simulink model "VRFB_lypunov_observer_model"  (R2024a)
settings: Solver=VariableStepAuto  StartTime=0.0  StopTime=10.0  RelTol=1e-3
undefined symbols (not defined in the file): c_V, d, E_neg, E_pos, E_T_23, E_T_34, E_T_45, eff_coulomb, F, g_neg, g_pos, gamma, H_init, k2, k3, k4, k5, kox, l, mu_init, R, S, T, u_upper_bound, Vc, Vt, x_real_init, z_13_low, z_13_up, z_24_low, z_24_up, z_hat_init
settings Model: Creator=DHADUKHA  LastModifiedBy=DHADUKHA

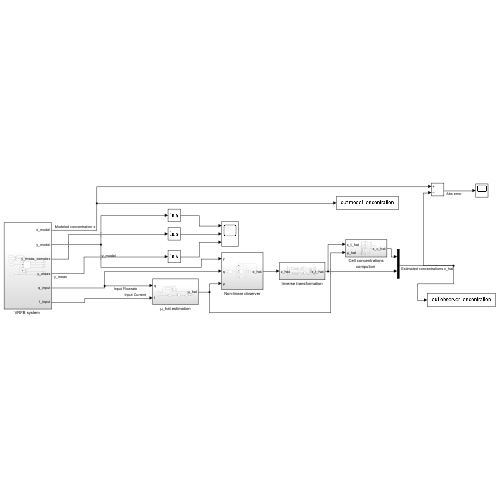
[thumbnail: Simulink's stored preview of the top-level diagram]
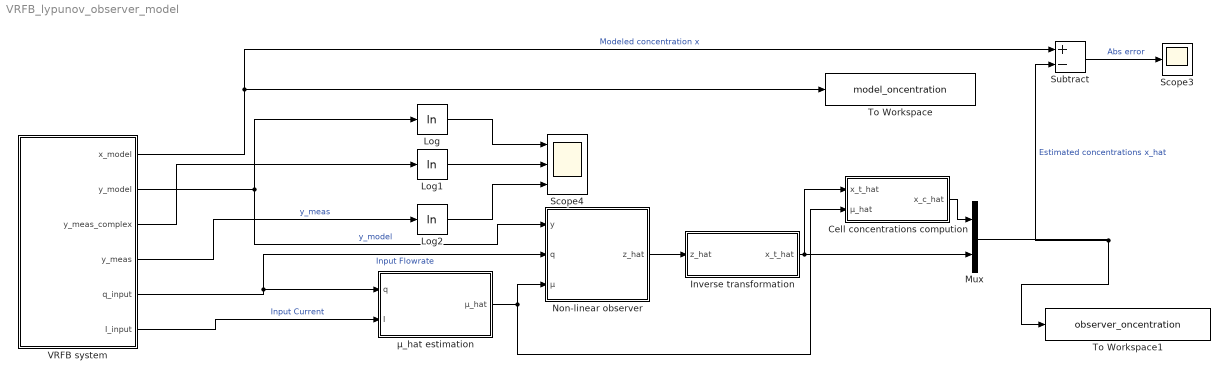
== system VRFB_lypunov_observer_model ==
  "Cell concentrations compution " : Subsystem
  "Inverse transformation " : Subsystem
  Log : Math  Operator=log
  Log1 : Math  Operator=log
  Log2 : Math  Operator=log
  Mux : Mux  Inputs=2
  "Non-linear observer " : Subsystem
  Scope3 : Scope
  Scope4 : Scope  NumInputPorts=3
  Subtract : Sum  Inputs=+-
  To Workspace : ToWorkspace  VariableName=model_oncentration  SaveFormat=Structure With Time  SampleTime=-1
  To Workspace1 : ToWorkspace  VariableName=observer_oncentration  SaveFormat=Structure With Time  SampleTime=-1
  "VRFB system " : Subsystem
  "µ_hat estimation " : Subsystem
  wires:
  "VRFB system "/5(q_input) -> "Non-linear observer "/2(q), "µ_hat estimation "/1(q)  "Input Flowrate"
  "VRFB system "/3(y_meas_complex) -> Log1/1
  "VRFB system "/1(x_model) -> Subtract/1, To Workspace/1  "Modeled concentration x"
  "VRFB system "/6(I_input) -> "µ_hat estimation "/2(I)  "Input Current"
  "VRFB system "/4(y_meas) -> Log2/1  "y_meas"
  "VRFB system "/2(y_model) -> "Non-linear observer "/1(y), Log/1  "y_model"
  Log1/1 -> Scope4/2
  Log/1 -> Scope4/1
  Log2/1 -> Scope4/3
  "µ_hat estimation "/1(µ_hat) -> "Non-linear observer "/3(µ), "Cell concentrations compution "/2(µ_hat)
  Subtract/1 -> Scope3/1  "Abs error"
  "Non-linear observer "/1(z_hat) -> "Inverse transformation "/1(z_hat)
  "Inverse transformation "/1(x_t_hat) -> "Cell concentrations compution "/1(x_t_hat), Mux/2
  "Cell concentrations compution "/1(x_c_hat) -> Mux/1
  Mux/1 -> Subtract/2, To Workspace1/1  "Estimated concentrations x_hat"

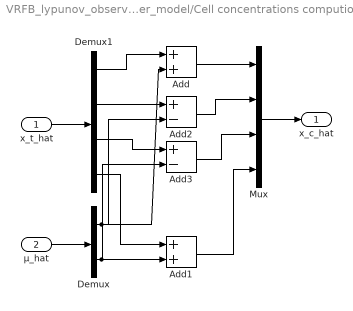
== system VRFB_lypunov_observer_model/Cell concentrations compution  ==
  x_t_hat : Inport
  µ_hat : Inport  Port=2
  Add : Sum
  Add1 : Sum
  Add2 : Sum  Inputs=+-
  Add3 : Sum  Inputs=+-
  Demux : Demux  Outputs=2
  Demux1 : Demux
  Mux : Mux
  x_c_hat : Outport
  wires:
  Demux1/4 -> Add1/1
  x_t_hat/1 -> Demux1/1
  Demux1/3 -> Add3/1
  µ_hat/1 -> Demux/1
  Demux/2 -> Add3/2, Add1/2
  Demux1/2 -> Add2/1
  Demux1/1 -> Add/1
  Demux/1 -> Add/2, Add2/2
  Add/1 -> Mux/1
  Add2/1 -> Mux/2
  Add3/1 -> Mux/3
  Add1/1 -> Mux/4
  Mux/1 -> x_c_hat/1

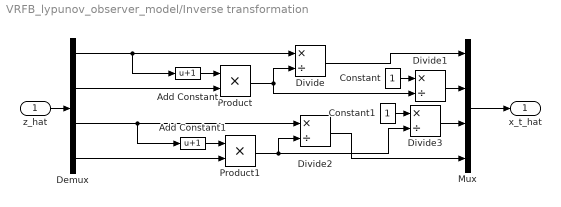
== system VRFB_lypunov_observer_model/Inverse transformation  ==
  z_hat : Inport
  Add Constant : Bias  Bias=1  SaturateOnIntegerOverflow=off
  Add Constant1 : Bias  Bias=1  SaturateOnIntegerOverflow=off
  Constant : Constant
  Constant1 : Constant
  Demux : Demux
  Divide{,1..3} (4 alike) : Product  Inputs=*/
  Mux : Mux
  Product : Product
  Product1 : Product
  x_t_hat : Outport
  wires:
  z_hat/1 -> Demux/1
  Demux/1 -> Add Constant/1, Divide/1
  Add Constant/1 -> Product/1
  Demux/2 -> Product/2
  Product/1 -> Divide1/2, Divide/2
  Mux/1 -> x_t_hat/1
  Divide/1 -> Mux/1
  Constant/1 -> Divide1/1
  Divide1/1 -> Mux/2
  Constant1/1 -> Divide3/1
  Product1/1 -> Divide2/2, Divide3/2
  Demux/4 -> Product1/2
  Add Constant1/1 -> Product1/1
  Demux/3 -> Divide2/1, Add Constant1/1
  Divide3/1 -> Mux/3
  Divide2/1 -> Mux/4

== system VRFB_lypunov_observer_model/Non-linear observer  ==
  y : Inport
  q : Inport  Port=2
  µ : Inport  Port=3
  Integrator : Integrator  InitialCondition=z_hat_init
  M(z_hat) : Subsystem
  Plus : Sum  Inputs=+++
  "f(z_hat, u)" : Subsystem
  "g(z_hat, y, u)" : Subsystem
  "u " : Subsystem
  z_hat : Outport
  wires:
  "f(z_hat, u)"/1(f) -> Plus/1
  "g(z_hat, y, u)"/1(g) -> Plus/2
  M(z_hat)/1(M) -> Plus/3
  Plus/1 -> Integrator/1  "z_hat_dot"
  Integrator/1 -> M(z_hat)/1(z_hat), "g(z_hat, y, u)"/1(z_hat), "f(z_hat, u)"/1(z_hat), z_hat/1
  q/1 -> "u "/1(q)
  "u "/1(u) -> M(z_hat)/2(u), "g(z_hat, y, u)"/3(u), "f(z_hat, u)"/2(u)
  y/1 -> "g(z_hat, y, u)"/2(y)
  µ/1 -> "u "/2(µ)

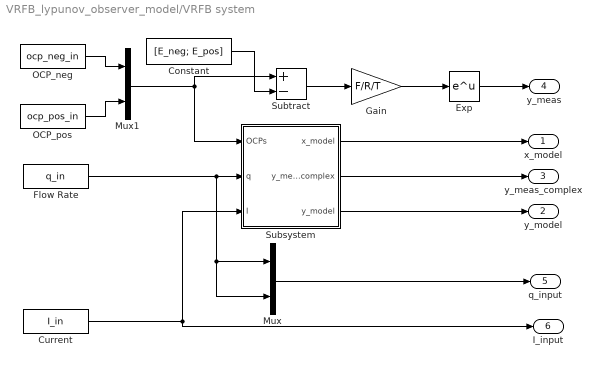
== system VRFB_lypunov_observer_model/VRFB system  ==
  Constant : Constant  Value=[E_neg; E_pos]
  Current : FromWorkspace  VariableName=I_in  SampleTime=1  OutputAfterFinalValue=Holding final value
  Exp : Math  OutputSignalType=real
  Flow Rate : FromWorkspace  VariableName=q_in  SampleTime=1  OutputAfterFinalValue=Holding final value
  Gain : Gain  Gain=F/R/T
  Mux : Mux  Inputs=2
  Mux1 : Mux  Inputs=2
  OCP_neg : FromWorkspace  VariableName=ocp_neg_in  SampleTime=1  OutputAfterFinalValue=Holding final value
  OCP_pos : FromWorkspace  VariableName=ocp_pos_in  SampleTime=1  OutputAfterFinalValue=Holding final value
  Subsystem : Subsystem
  Subtract : Sum  Inputs=+-
  x_model : Outport
  y_model : Outport  Port=2
  y_meas_complex : Outport  Port=3
  y_meas : Outport  Port=4
  q_input : Outport  Port=5
  I_input : Outport  Port=6
  wires:
  Subsystem/2(y_meas_complex) -> y_meas_complex/1
  Mux1/1 -> Subtract/1, Subsystem/1(OCPs)
  OCP_neg/1 -> Mux1/1
  Subsystem/1(x_model) -> x_model/1
  Flow Rate/1 -> Mux/1, Mux/2, Subsystem/2(q)
  Subtract/1 -> Gain/1
  OCP_pos/1 -> Mux1/2
  Current/1 -> Subsystem/3(I), I_input/1
  Constant/1 -> Subtract/2
  Subsystem/3(y_model) -> y_model/1
  Mux/1 -> q_input/1
  Gain/1 -> Exp/1
  Exp/1 -> y_meas/1

== system VRFB_lypunov_observer_model/µ_hat estimation  ==
  q : Inport
  I : Inport  Port=2
  Constant : Constant  Value=-(1/Vc+1/Vt)
  Gain : Gain  Gain=1/(F*Vc)
  Integrator : Integrator  InitialCondition=mu_init
  Plus : Sum
  Product : Product  Inputs=3
  µ_hat : Outport
  wires:
  I/1 -> Gain/1
  Gain/1 -> Plus/2
  q/1 -> Product/1
  Constant/1 -> Product/2
  Integrator/1 -> Product/3, µ_hat/1
  Product/1 -> Plus/1
  Plus/1 -> Integrator/1  "µ_dot_hat"

== system VRFB_lypunov_observer_model/Non-linear observer /M(z_hat) ==
  z_hat : Inport
  u : Inport  Port=2
  Constant1 : Constant  Value=[z_13_low; z_24_low; z_13_low; z_24_low]  VectorParams1D=off
  Constant2 : Constant  Value=[z_13_up; z_24_up; z_13_up; z_24_up]  VectorParams1D=off
  Gain : Gain  Gain=-gamma
  MATLAB Function : MATLAB Function  TreatAsAtomicUnit=on
  P-Matrix [4,4] : Subsystem
  Product : Product  Inputs=3  Multiplication=Matrix(*)
  "r(z_hat) " : Subsystem
  M : Outport
  wires:
  u/1 -> P-Matrix [4,4]/1(u)
  z_hat/1 -> MATLAB Function/1(z), "r(z_hat) "/1(z_hat)
  Constant2/1 -> MATLAB Function/3(z_max)
  Constant1/1 -> MATLAB Function/2(z_min)
  Product/1 -> Gain/1
  Gain/1 -> M/1
  P-Matrix [4,4]/1(P) -> Product/1
  MATLAB Function/1(drdz) -> Product/2
  "r(z_hat) "/1(r) -> Product/3

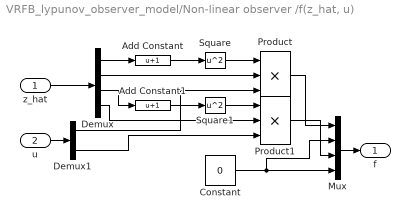
== system VRFB_lypunov_observer_model/Non-linear observer /f(z_hat, u) ==
  z_hat : Inport
  u : Inport  Port=2
  Add Constant : Bias  Bias=1  SaturateOnIntegerOverflow=off
  Add Constant1 : Bias  Bias=1  SaturateOnIntegerOverflow=off
  Constant : Constant  Value=0
  Demux : Demux
  Demux1 : Demux  Outputs=2
  Mux : Mux
  Product : Product  Inputs=3
  Product1 : Product  Inputs=3
  Square : Math  Operator=square
  Square1 : Math  Operator=square
  f : Outport
  wires:
  z_hat/1 -> Demux/1
  Mux/1 -> f/1
  Constant/1 -> Mux/2, Mux/4
  u/1 -> Demux1/1
  Demux/1 -> Add Constant/1
  Add Constant/1 -> Square/1
  Square/1 -> Product/1
  Demux1/1 -> Product/3
  Demux/2 -> Product/2
  Add Constant1/1 -> Square1/1
  Square1/1 -> Product1/1
  Demux/4 -> Product1/2
  Demux1/2 -> Product1/3
  Demux/3 -> Add Constant1/1
  Product1/1 -> Mux/3
  Product/1 -> Mux/1

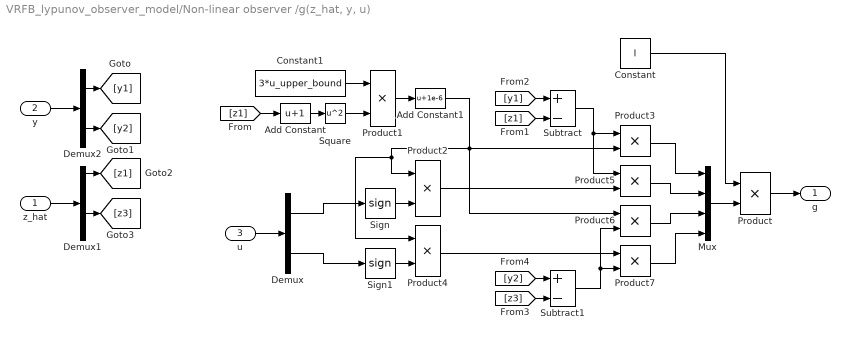
== system VRFB_lypunov_observer_model/Non-linear observer /g(z_hat, y, u) ==
  z_hat : Inport
  y : Inport  Port=2
  u : Inport  Port=3
  Add Constant : Bias  Bias=1  SaturateOnIntegerOverflow=off
  Add Constant1 : Bias  Bias=1e-6  SaturateOnIntegerOverflow=off
  Constant : Constant  Value=l
  Constant1 : Constant  Value=3*u_upper_bound
  Demux : Demux  Outputs=2
  Demux1 : Demux
  Demux2 : Demux  Outputs=2
  Mux : Mux
  Product{,1..7} (8 alike) : Product
  Sign : Signum
  Sign1 : Signum
  Square : Math  Operator=square
  Subtract : Sum  Inputs=+-
  Subtract1 : Sum  Inputs=+-
  g : Outport
  wires:
  u/1 -> Demux/1
  z_hat/1 -> Demux1/1
  y/1 -> Demux2/1
  Product/1 -> g/1
  Mux/1 -> Product/2
  Constant/1 -> Product/1
  Add Constant/1 -> Square/1
  Constant1/1 -> Product1/1
  Square/1 -> Product1/2
  Demux2/1 -> [y1]
  Demux2/2 -> [y2]
  Demux1/1 -> [z1]
  Demux1/3 -> [z3]
  [z1] -> Add Constant/1
  Product1/1 -> Add Constant1/1
  Demux/1 -> Sign/1
  Demux/2 -> Sign1/1
  Product2/1 -> Product5/2
  Product4/1 -> Product7/1
  Sign/1 -> Product2/2
  Add Constant1/1 -> Product6/1, Product2/1, Product4/1, Product3/2
  Sign1/1 -> Product4/2
  [z1] -> Subtract/2
  [y1] -> Subtract/1
  [z3] -> Subtract1/2
  [y2] -> Subtract1/1
  Product6/1 -> Mux/3
  Product5/1 -> Mux/2
  Product3/1 -> Mux/1
  Product7/1 -> Mux/4
  Subtract/1 -> Product5/1, Product3/1
  Subtract1/1 -> Product6/2, Product7/2

== system VRFB_lypunov_observer_model/Non-linear observer /u  ==
  q : Inport
  µ : Inport  Port=2
  Constant : Constant  Value=Vt
  Divide1 : Product  Inputs=**/
  u : Outport
  wires:
  Divide1/1 -> u/1  "u"
  Constant/1 -> Divide1/3
  q/1 -> Divide1/1
  µ/1 -> Divide1/2

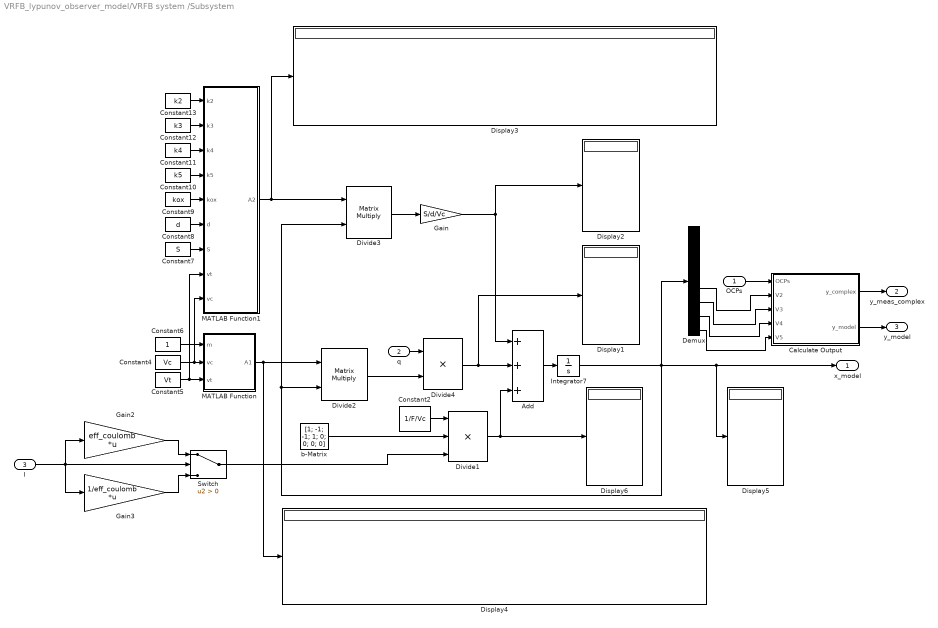
== system VRFB_lypunov_observer_model/VRFB system /Subsystem ==
  OCPs : Inport
  q : Inport  Port=2
  I : Inport  Port=3
  Add : Sum  Inputs=+++
  Calculate Output : Subsystem
  Constant10 : Constant  Value=k5
  Constant11 : Constant  Value=k4
  Constant12 : Constant  Value=k3
  Constant13 : Constant  Value=k2
  Constant2 : Constant  Value=1/F/Vc
  Constant4 : Constant  Value=Vc
  Constant5 : Constant  Value=Vt
  Constant6 : Constant
  Constant7 : Constant  Value=S
  Constant8 : Constant  Value=d
  Constant9 : Constant  Value=kox
  Demux : Demux  Outputs=8
  Display{1..6} (6 alike) : Display
  Divide1 : Product  Inputs=***
  Divide2 : Product  Inputs=**  Multiplication=Matrix(*)
  Divide3 : Product  Inputs=**  Multiplication=Matrix(*)
  Divide4 : Product  Inputs=**
  Gain : Gain  Gain=S/d/Vc
  Gain2 : Gain  Gain=eff_coulomb  Multiplication=Matrix(K*u)
  Gain3 : Gain  Gain=1/eff_coulomb  Multiplication=Matrix(K*u)
  Integrator7 : Integrator  InitialCondition=x_real_init
  MATLAB Function : MATLAB Function  TreatAsAtomicUnit=on
  MATLAB Function1 : MATLAB Function  TreatAsAtomicUnit=on
  Switch : Switch  Criteria=u2 > Threshold  SaturateOnIntegerOverflow=off  InputSameDT=off
  b-Matrix : Constant  Value=[1; -1; -1; 1; 0; 0; 0; 0]
  x_model : Outport
  y_meas_complex : Outport  Port=2
  y_model : Outport  Port=3
  wires:
  Integrator7/1 -> Display5/1, x_model/1, Divide3/2, Divide2/2, Demux/1
  b-Matrix/1 -> Divide1/2
  Constant2/1 -> Divide1/1
  Divide1/1 -> Display6/1, Add/3
  Constant4/1 -> MATLAB Function1/9(vc), MATLAB Function/2(vc)
  Constant5/1 -> MATLAB Function1/8(vt), MATLAB Function/3(vt)
  Constant6/1 -> MATLAB Function/1(m)
  Constant13/1 -> MATLAB Function1/1(k2)
  Constant12/1 -> MATLAB Function1/2(k3)
  Constant11/1 -> MATLAB Function1/3(k4)
  Constant10/1 -> MATLAB Function1/4(k5)
  Constant9/1 -> MATLAB Function1/5(kox)
  Constant8/1 -> MATLAB Function1/6(d)
  Constant7/1 -> MATLAB Function1/7(S)
  MATLAB Function1/1(A2) -> Divide3/1, Display3/1
  Add/1 -> Integrator7/1
  Divide3/1 -> Gain/1
  Gain/1 -> Display2/1, Add/1
  q/1 -> Divide4/1
  Divide2/1 -> Divide4/2
  Divide4/1 -> Add/2, Display1/1
  MATLAB Function/1(A1) -> Display4/1, Divide2/1
  Gain2/1 -> Switch/1
  Gain3/1 -> Switch/3
  I/1 -> Gain2/1, Gain3/1, Switch/2
  Switch/1 -> Divide1/3
  Demux/6 -> Calculate Output/3(V3)
  Demux/7 -> Calculate Output/4(V4)
  Demux/8 -> Calculate Output/5(V5)
  OCPs/1 -> Calculate Output/1(OCPs)
  Demux/5 -> Calculate Output/2(V2)
  Calculate Output/1(y_complex) -> y_meas_complex/1
  Calculate Output/2(y_model) -> y_model/1

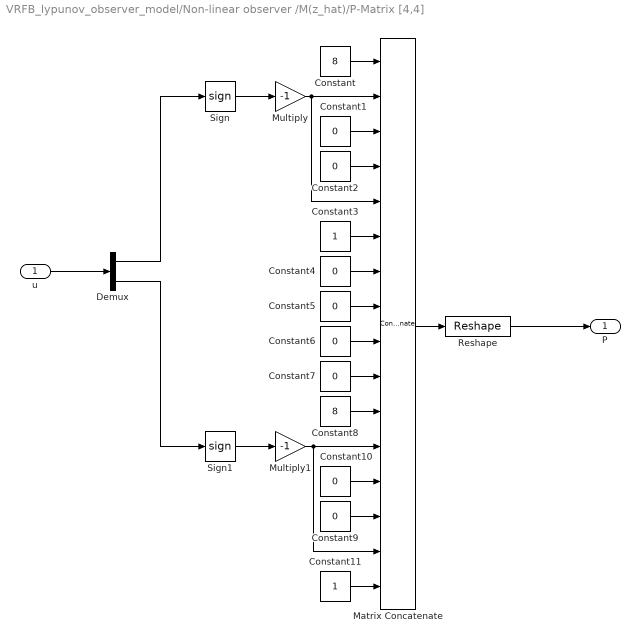
== system VRFB_lypunov_observer_model/Non-linear observer /M(z_hat)/P-Matrix [4,4] ==
  u : Inport
  Constant : Constant  Value=8
  Constant{1..2,4..7,9..10} (8 alike) : Constant  Value=0
  Constant11 : Constant
  Constant3 : Constant
  Constant8 : Constant  Value=8
  Demux : Demux  Outputs=2
  Matrix Concatenate : Concatenate  NumInputs=16  ConcatenateDimension=2
  Multiply : Gain  Gain=-1
  Multiply1 : Gain  Gain=-1
  Reshape : Reshape  OutputDimensionality=Customize  OutputDimensions=[4,4]
  Sign : Signum
  Sign1 : Signum
  P : Outport
  wires:
  Reshape/1 -> P/1
  Constant10/1 -> Matrix Concatenate/13
  Constant11/1 -> Matrix Concatenate/16
  Constant4/1 -> Matrix Concatenate/7
  Sign1/1 -> Multiply1/1
  Sign/1 -> Multiply/1
  u/1 -> Demux/1
  Demux/2 -> Sign1/1
  Constant8/1 -> Matrix Concatenate/11
  Constant3/1 -> Matrix Concatenate/6
  Multiply/1 -> Matrix Concatenate/5, Matrix Concatenate/2
  Constant6/1 -> Matrix Concatenate/9
  Constant7/1 -> Matrix Concatenate/10
  Constant5/1 -> Matrix Concatenate/8
  Matrix Concatenate/1 -> Reshape/1
  Constant2/1 -> Matrix Concatenate/4
  Constant1/1 -> Matrix Concatenate/3
  Multiply1/1 -> Matrix Concatenate/15, Matrix Concatenate/12
  Constant9/1 -> Matrix Concatenate/14
  Demux/1 -> Sign/1
  Constant/1 -> Matrix Concatenate/1

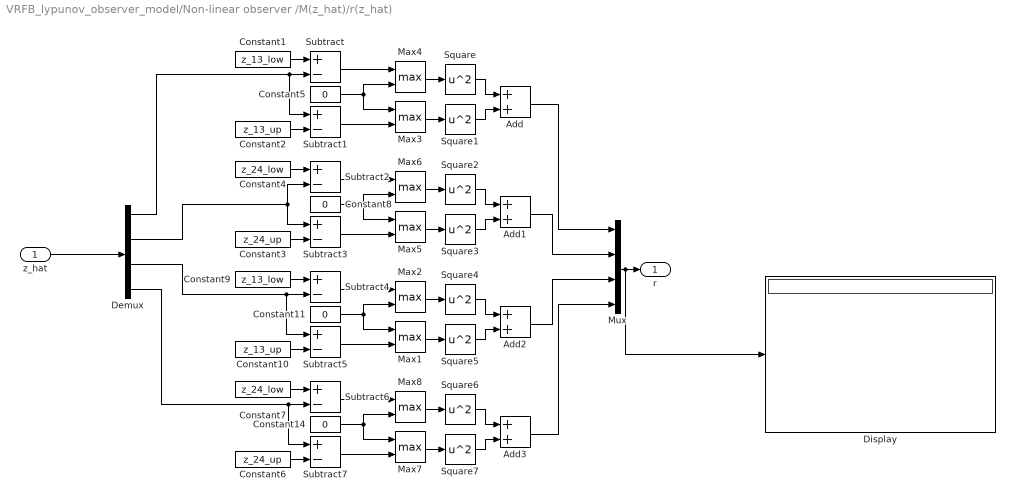
== system VRFB_lypunov_observer_model/Non-linear observer /M(z_hat)/r(z_hat)  ==
  z_hat : Inport
  Add{,1..3} (4 alike) : Sum
  Constant1 : Constant  Value=z_13_low
  Constant10 : Constant  Value=z_13_up
  Constant{5,8,11,14} (4 alike) : Constant  Value=0
  Constant2 : Constant  Value=z_13_up
  Constant3 : Constant  Value=z_24_up
  Constant4 : Constant  Value=z_24_low
  Constant6 : Constant  Value=z_24_up
  Constant7 : Constant  Value=z_24_low
  Constant9 : Constant  Value=z_13_low
  Demux : Demux
  Display : Display
  Max{1..8} (8 alike) : MinMax  Function=max  Inputs=2
  Mux : Mux
  Square{,1..7} (8 alike) : Math  Operator=square
  Subtract{,1..7} (8 alike) : Sum  Inputs=+-
  r : Outport
  wires:
  Mux/1 -> Display/1, r/1
  Max2/1 -> Square4/1
  Constant6/1 -> Subtract7/2
  Max8/1 -> Square6/1
  Max1/1 -> Square5/1
  Square4/1 -> Add2/1
  Add3/1 -> Mux/4
  Square3/1 -> Add1/2
  Subtract2/1 -> Max6/1
  Subtract1/1 -> Max3/2
  Constant10/1 -> Subtract5/2
  Subtract3/1 -> Max5/2
  Square6/1 -> Add3/1
  Constant7/1 -> Subtract6/1
  Max6/1 -> Square2/1
  Square2/1 -> Add1/1
  Constant3/1 -> Subtract3/2
  Constant9/1 -> Subtract4/1
  Subtract5/1 -> Max1/2
  Square/1 -> Add/1
  Max5/1 -> Square3/1
  Max4/1 -> Square/1
  Subtract7/1 -> Max7/2
  Square5/1 -> Add2/2
  z_hat/1 -> Demux/1
  Constant11/1 -> Max2/2, Max1/1
  Subtract6/1 -> Max8/1
  Subtract4/1 -> Max2/1
  Constant2/1 -> Subtract1/2
  Subtract/1 -> Max4/1
  Demux/4 -> Subtract7/1, Subtract6/2
  Add/1 -> Mux/1
  Max7/1 -> Square7/1
  Demux/3 -> Subtract5/1, Subtract4/2
  Constant5/1 -> Max4/2, Max3/1
  Constant8/1 -> Max6/2, Max5/1
  Square1/1 -> Add/2
  Constant14/1 -> Max8/2, Max7/1
  Constant1/1 -> Subtract/1
  Demux/2 -> Subtract2/2, Subtract3/1
  Add2/1 -> Mux/3
  Square7/1 -> Add3/2
  Max3/1 -> Square1/1
  Add1/1 -> Mux/2
  Demux/1 -> Subtract1/1, Subtract/2
  Constant4/1 -> Subtract2/1

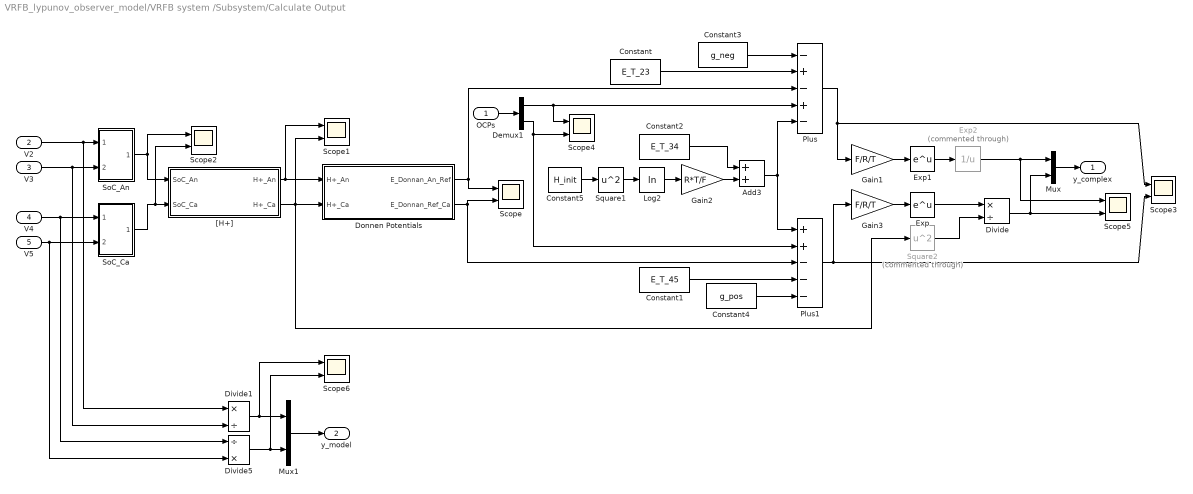
== system VRFB_lypunov_observer_model/VRFB system /Subsystem/Calculate Output ==
  OCPs : Inport
  V2 : Inport  Port=2
  V3 : Inport  Port=3
  V4 : Inport  Port=4
  V5 : Inport  Port=5
  Add3 : Sum
  Constant : Constant  Value=E_T_23
  Constant1 : Constant  Value=E_T_45
  Constant2 : Constant  Value=E_T_34
  Constant3 : Constant  Value=g_neg
  Constant4 : Constant  Value=g_pos
  Constant5 : Constant  Value=H_init
  Demux1 : Demux  Outputs=2
  Divide : Product  Inputs=*/
  Divide1 : Product  Inputs=*/
  Divide5 : Product  Inputs=/*
  Donnen Potentials : Subsystem
  Exp : Math
  Exp1 : Math
  Exp2 : Math  Commented=through  Operator=reciprocal
  Gain1 : Gain  Gain=F/R/T
  Gain2 : Gain  Gain=R*T/F
  Gain3 : Gain  Gain=F/R/T
  Log2 : Math  Operator=log
  Mux : Mux  Inputs=2
  Mux1 : Mux  Inputs=2
  Plus : Sum  Inputs=-+-+-
  Plus1 : Sum  Inputs=++---
  Scope{,1..6} (7 alike) : Scope  NumInputPorts=2
  SoC_An : Subsystem
  SoC_Ca : Subsystem
  Square1 : Math  Operator=square
  Square2 : Math  Commented=through  Operator=square
  "[H+]" : Subsystem
  y_complex : Outport
  y_model : Outport  Port=2
  wires:
  OCPs/1 -> Demux1/1
  Plus/1 -> Gain1/1, Scope3/1
  Plus1/1 -> Gain3/1, Scope3/2
  SoC_An/1(Out1) -> Scope2/1, "[H+]"/1(SoC_An)
  SoC_Ca/1(Out1) -> Scope2/2, "[H+]"/2(SoC_Ca)
  "[H+]"/1(H+_An) -> Scope1/1, Donnen Potentials/1(H+_An)
  "[H+]"/2(H+_Ca) -> Scope1/2, Square2/1, Donnen Potentials/2(H+_Ca)
  Donnen Potentials/2(E_Donnan_Ref_Ca) -> Scope/2, Plus1/3
  Constant/1 -> Plus/2
  Donnen Potentials/1(E_Donnan_An_Ref) -> Plus/3, Scope/1
  Constant4/1 -> Plus1/5
  Constant3/1 -> Plus/1
  Gain2/1 -> Add3/2
  Log2/1 -> Gain2/1
  Constant2/1 -> Add3/1
  Demux1/1 -> Scope4/1, Plus/4
  Demux1/2 -> Scope4/2, Plus1/2
  Add3/1 -> Plus1/1, Plus/5
  Gain3/1 -> Exp/1
  Constant5/1 -> Square1/1
  Square1/1 -> Log2/1
  Constant1/1 -> Plus1/4
  Mux/1 -> y_complex/1
  Gain1/1 -> Exp1/1
  Square2/1 -> Divide/2
  Exp/1 -> Divide/1
  Divide/1 -> Scope5/2, Mux/2
  Exp1/1 -> Exp2/1
  Exp2/1 -> Scope5/1, Mux/1
  Divide5/1 -> Scope6/2, Mux1/2
  V2/1 -> Divide1/1, SoC_An/1(In1)
  V4/1 -> Divide5/1, SoC_Ca/1(In1)
  Divide1/1 -> Scope6/1, Mux1/1
  Mux1/1 -> y_model/1
  V5/1 -> Divide5/2, SoC_Ca/2(In2)
  V3/1 -> Divide1/2, SoC_An/2(In2)

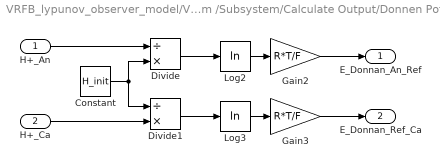
== system VRFB_lypunov_observer_model/VRFB system /Subsystem/Calculate Output/Donnen Potentials ==
  H+_An : Inport
  H+_Ca : Inport  Port=2
  Constant : Constant  Value=H_init
  Divide : Product  Inputs=/*
  Divide1 : Product  Inputs=/*
  Gain2 : Gain  Gain=R*T/F
  Gain3 : Gain  Gain=R*T/F
  Log2 : Math  Operator=log
  Log3 : Math  Operator=log
  E_Donnan_An_Ref : Outport
  E_Donnan_Ref_Ca : Outport  Port=2
  wires:
  H+_An/1 -> Divide/1
  Gain3/1 -> E_Donnan_Ref_Ca/1
  Gain2/1 -> E_Donnan_An_Ref/1
  H+_Ca/1 -> Divide1/2
  Log3/1 -> Gain3/1
  Divide/1 -> Log2/1
  Divide1/1 -> Log3/1
  Log2/1 -> Gain2/1
  Constant/1 -> Divide/2, Divide1/1

== system VRFB_lypunov_observer_model/VRFB system /Subsystem/Calculate Output/SoC_An ==
  In1 : Inport
  In2 : Inport  Port=2
  Add3 : Sum
  Divide1 : Product  Inputs=*/
  Out1 : Outport
  wires:
  Divide1/1 -> Out1/1
  In1/1 -> Add3/1, Divide1/1
  Add3/1 -> Divide1/2
  In2/1 -> Add3/2

== system VRFB_lypunov_observer_model/VRFB system /Subsystem/Calculate Output/SoC_Ca ==
  In1 : Inport
  In2 : Inport  Port=2
  Add4 : Sum
  Divide : Product  Inputs=*/
  Out1 : Outport
  wires:
  Add4/1 -> Divide/2
  In1/1 -> Add4/1
  Divide/1 -> Out1/1
  In2/1 -> Divide/1, Add4/2

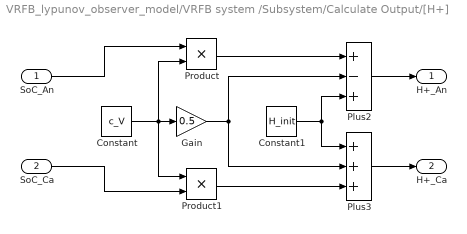
== system VRFB_lypunov_observer_model/VRFB system /Subsystem/Calculate Output/[H+] ==
  SoC_An : Inport
  SoC_Ca : Inport  Port=2
  Constant : Constant  Value=c_V
  Constant1 : Constant  Value=H_init
  Gain : Gain  Gain=0.5
  Plus2 : Sum  Inputs=+-+
  Plus3 : Sum  Inputs=+++
  Product : Product
  Product1 : Product
  H+_An : Outport
  H+_Ca : Outport  Port=2
  wires:
  Plus3/1 -> H+_Ca/1
  SoC_Ca/1 -> Product1/2
  Product1/1 -> Plus3/3
  Constant1/1 -> Plus2/3, Plus3/1
  Product/1 -> Plus2/1
  Gain/1 -> Plus2/2, Plus3/2
  Plus2/1 -> H+_An/1
  SoC_An/1 -> Product/1
  Constant/1 -> Product1/1, Product/2, Gain/1

== matlab function VRFB_lypunov_observer_model/VRFB system /Subsystem/MATLAB Function ==
  data: m input; A1 output; vc input; vt input
function A1 = A1_full(m, vc, vt)
% Returns the full 8x8 A1 matrix (Appendix A.1 of the paper)
% m: membrane porosity factor
% vc: cell volume
% vt: tank volume

    A1 = zeros(8,8);

    a = 1 / (m * vc);
    b = 1 / vt;

    % Negative side (cell to tank coupling)
    A1(1,1) = -a;
    A1(2,2) = -a;
    A1(3,3) = -a;
    A1(4,4) = -a;
    A1(1,5) = a;
    A1(2,6) = a;
    A1(3,7) = a;
    A1(4,8) = a;

    % Tank dynamics (positive diagonal, negative off-diagonal)
    A1(5,5) = -b;
    A1(6,6) = -b;
    A1(7,7) = -b;
    A1(8,8) = -b;
    A1(5,1) = b;
    A1(6,2) = b;
    A1(7,3) = b;
    A1(8,4) = b;
end

== matlab function VRFB_lypunov_observer_model/Non-linear observer /M(z_hat)/MATLAB Function ==
  data: z input; drdz output; z_min input; z_max input
function drdz = projection_jacobian(z, z_min, z_max)
    % Computes the partial derivative dr/dz for the projection correction term

    drdz = zeros(4,4);
    for i = 1:4
        if z(i) > z_max(i)
            drdz(i,i) = 2 * (z(i) - z_max(i));
        elseif z(i) < z_min(i)
            drdz(i,i) = 2 * (z(i) - z_min(i));  % this is correct, not z_min - z(i)
        else
            drdz(i,i) = 0;
        end
    end
end

== matlab function VRFB_lypunov_observer_model/VRFB system /Subsystem/MATLAB Function1 ==
  data: k2 input; A2 output; k3 input; k4 input; k5 input; kox input; d input; S input; vt input; vc input
function A2 = A2_full(k2, k3, k4, k5, kox, d, S, vt, vc)
% Returns the full 8x8 A2 matrix (Appendix A.1 of the paper)
% k2 to k5: chemical reaction rate constants
% kox: oxygen side reaction rate
% d, S: electrode thickness and area
% vt, vc: tank and cell volumes

    A2 = zeros(8,8);

    % Chemical reactions in cells
    A2(1,1) = -k2;
    A2(1,3) = -k4;
    A2(1,4) = -2*k5;

    A2(2,2) = -k3;
    A2(2,3) = 2*k4;
    A2(2,4) = 3*k5;

    A2(3,1) = 3*k2;
    A2(3,2) = 2*k3;
    A2(3,3) = -k4;

    A2(4,1) = -2*k2;
    A2(4,2) = -k3;
    A2(4,4) = -k5;

    % Side reactions in cells (oxygen evolution at cathode)
    scale = kox * d * S / (vt * vc);
    A2(5,5) = -scale;
    A2(6,6) =  scale;

    % No dynamics defined for x7 and x8 in A2
end
